simulink model "modulator"  (R2025b)
settings: Solver=ode23tb  StartTime=0.0  StopTime=simlength  FixedStep=tc  MaxStep=tc
undefined symbols (not defined in the file): freq, tc, ts_afe
libraries: SV_pattern_generator_with_global_TRGO x4
settings Model: Creator=dbagn  LastModifiedBy=dbagn
settings SolverCC: NumberNewtonIterations=3.0  ZeroCrossControl=DisableAll  AlgebraicLoopSolver=TrustRegion  SolverResetMethod=Robust
settings DataIOCC: ReturnWorkspaceOutputs=off
settings OptimizationCC: ReuseModelBlockBuffer=off
settings DebuggingCC: UnconnectedInputMsg=warning  UnconnectedOutputMsg=warning  UnconnectedLineMsg=warning
settings ModelReferenceCC: EnableRefExpFcnMdlSchedulingChecks=on
settings SFSimCC: CustomCodeUndefinedFunction=ThrowError
settings SFSimCC: SimCustomHeaderCode=|
  | #include "math_f.h"
  | #include "mavgflt.h"
  | #include "mavgflt_simulink.h"
  | #include "bemf_obsv.h"
  | #include "bemf_obsv_simulink.h"
  | #include "bemf_obsv_load_est.h"
  | #include "bemf_obsv_load_est_simulink.h"
  | #include "dqvector_pi.h"
  | #include "dqvector_pi_simulink.h"
  | #include "sv_pwm_simulink.h"
  | #include "sv_pwm.h"
settings SFSimCC: SimUserSources=|
  | "mavgflt_simulink.c"
  | "mavgflt.c"
  | "bemf_obsv_simulink.c"
  | "bemf_obsv.c"
  | "bemf_obsv_load_est_simulink.c"
  | "bemf_obsv_load_est.c"
  | "dqvector_pi.c"
  | "dqvector_pi_simulink.c"
  | "sv_pwm_simulink.c"
  | "sv_pwm.c"
settings SFSimCC: SimUserIncludeDirs=|
  | include
  | src
settings RTWCC: GPUComputeCapability=3.5  DLArmComputeVersion=19.05

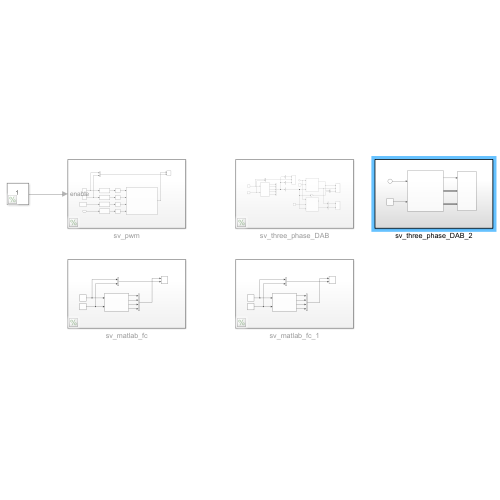
[thumbnail: Simulink's stored preview of the top-level diagram]
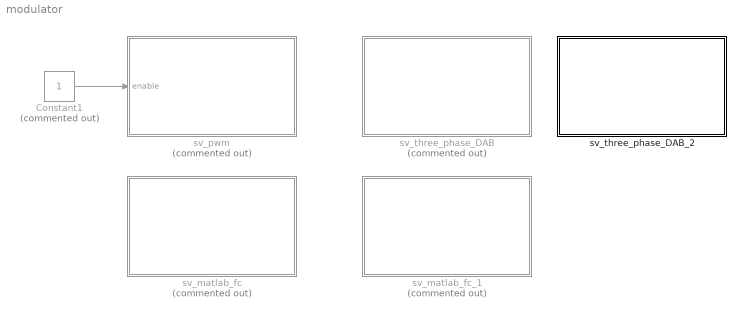
== system modulator ==
  Constant1 : Constant  Commented=on
  sv_matlab_fc : Subsystem  Commented=on
  sv_matlab_fc_1 : Subsystem  Commented=on
  sv_pwm : Subsystem  Commented=on
  sv_three_phase_DAB : Subsystem  Commented=on
  sv_three_phase_DAB_2 : Subsystem
  wires:
  Constant1/1 -> sv_pwm/1(enable)

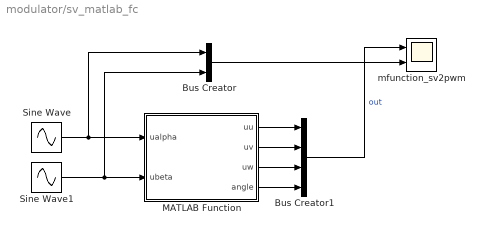
== system modulator/sv_matlab_fc ==
  Bus Creator : BusCreator  Inputs=2
  Bus Creator1 : BusCreator  Inputs=4
  MATLAB Function : MATLAB Function  TreatAsAtomicUnit=on  SystemSampleTime=ts_afe
  Sine Wave : Sin  Amplitude=sqrt(3)/2  Frequency=2*pi*50  SampleTime=0
  Sine Wave1 : Sin  Amplitude=sqrt(3)/2  Frequency=2*pi*50  Phase=-pi/2  SampleTime=0
  mfunction_sv2pwm : Scope  NumInputPorts=2
      settings: ActiveDisplayYMinimum=-3.9269908169872405  ActiveDisplayYMaximum=3.9269908169872392
  wires:
  Bus Creator/1 -> mfunction_sv2pwm/2
  Bus Creator1/1 -> mfunction_sv2pwm/1  "out"
  Sine Wave1/1 -> MATLAB Function/2(ubeta), Bus Creator/2
  Sine Wave/1 -> MATLAB Function/1(ualpha), Bus Creator/1
  MATLAB Function/3(uw) -> Bus Creator1/3
  MATLAB Function/2(uv) -> Bus Creator1/2
  MATLAB Function/1(uu) -> Bus Creator1/1
  MATLAB Function/4(angle) -> Bus Creator1/4

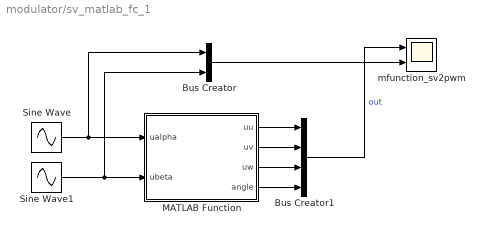
== system modulator/sv_matlab_fc_1 ==
  Bus Creator : BusCreator  Inputs=2
  Bus Creator1 : BusCreator  Inputs=4
  MATLAB Function : MATLAB Function  TreatAsAtomicUnit=on  SystemSampleTime=ts_afe
  Sine Wave : Sin  Amplitude=sqrt(3)/2  Frequency=2*pi*50  SampleTime=0
  Sine Wave1 : Sin  Amplitude=sqrt(3)/2  Frequency=2*pi*50  Phase=-pi/2  SampleTime=0
  mfunction_sv2pwm : Scope  NumInputPorts=2
      settings: ActiveDisplayYMinimum=-0.785398163397448  ActiveDisplayYMaximum=7.0685834705770336
  wires:
  MATLAB Function/4(angle) -> Bus Creator1/4
  MATLAB Function/1(uu) -> Bus Creator1/1
  MATLAB Function/2(uv) -> Bus Creator1/2
  MATLAB Function/3(uw) -> Bus Creator1/3
  Sine Wave/1 -> Bus Creator/1, MATLAB Function/1(ualpha)
  Sine Wave1/1 -> Bus Creator/2, MATLAB Function/2(ubeta)
  Bus Creator1/1 -> mfunction_sv2pwm/1  "out"
  Bus Creator/1 -> mfunction_sv2pwm/2

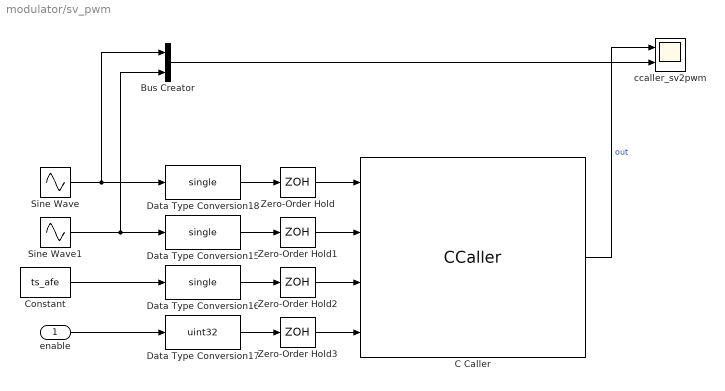
== system modulator/sv_pwm ==
  enable : Inport
  Bus Creator : BusCreator  Inputs=2
  C Caller : CCaller  FunctionName=sv_pwm_process_simulink  PortSpecificationStruct="%)30     .    V @   8    (     @         %    \"     4    !     0         %  0 \"0    $    _    07)G3F%M90  4&]R=$YA;64 4V-O<&4     26YD97@     5'EP90      4VEZ90      27-';&]B86P   X    P    !@    @    $          4    (     0    ,    !         !   P!O=70 #@   #     &    \"     0         !0    @    !     P    $         $  # &]U=  .    .     8    (    !          %    \"     $    &     0         0   ...(+2669 chars)"  SampleTime=ts_afe
  Constant : Constant  Value=ts_afe
  Data Type Conversion15 : DataTypeConversion  OutDataTypeStr=single  SaturateOnIntegerOverflow=off  RndMeth=Floor
  Data Type Conversion16 : DataTypeConversion  OutDataTypeStr=single  SaturateOnIntegerOverflow=off  RndMeth=Floor
  Data Type Conversion17 : DataTypeConversion  OutDataTypeStr=uint32  SaturateOnIntegerOverflow=off  RndMeth=Floor
  Data Type Conversion18 : DataTypeConversion  OutDataTypeStr=single  SaturateOnIntegerOverflow=off  RndMeth=Floor
  Sine Wave : Sin  Amplitude=sqrt(3)/2  Frequency=2*pi*50  SampleTime=0
  Sine Wave1 : Sin  Amplitude=sqrt(3)/2  Frequency=2*pi*50  Phase=pi/2  SampleTime=0
  Zero-Order Hold{,1..3} (4 alike) : ZeroOrderHold  SampleTime=ts_afe
  ccaller_sv2pwm : Scope  NumInputPorts=2
      settings: SampleTime=ts_afe  ActiveDisplayYMinimum=-0.54922  ActiveDisplayYMaximum=1.54922
  wires:
  Zero-Order Hold2/1 -> C Caller/3
  Constant/1 -> Data Type Conversion16/1
  Data Type Conversion18/1 -> Zero-Order Hold/1
  enable/1 -> Data Type Conversion17/1
  Data Type Conversion16/1 -> Zero-Order Hold2/1
  Data Type Conversion17/1 -> Zero-Order Hold3/1
  Zero-Order Hold3/1 -> C Caller/4
  Data Type Conversion15/1 -> Zero-Order Hold1/1
  Zero-Order Hold/1 -> C Caller/1
  Zero-Order Hold1/1 -> C Caller/2
  C Caller/1 -> ccaller_sv2pwm/1  "out"
  Sine Wave/1 -> Bus Creator/1, Data Type Conversion18/1
  Sine Wave1/1 -> Bus Creator/2, Data Type Conversion15/1
  Bus Creator/1 -> ccaller_sv2pwm/2

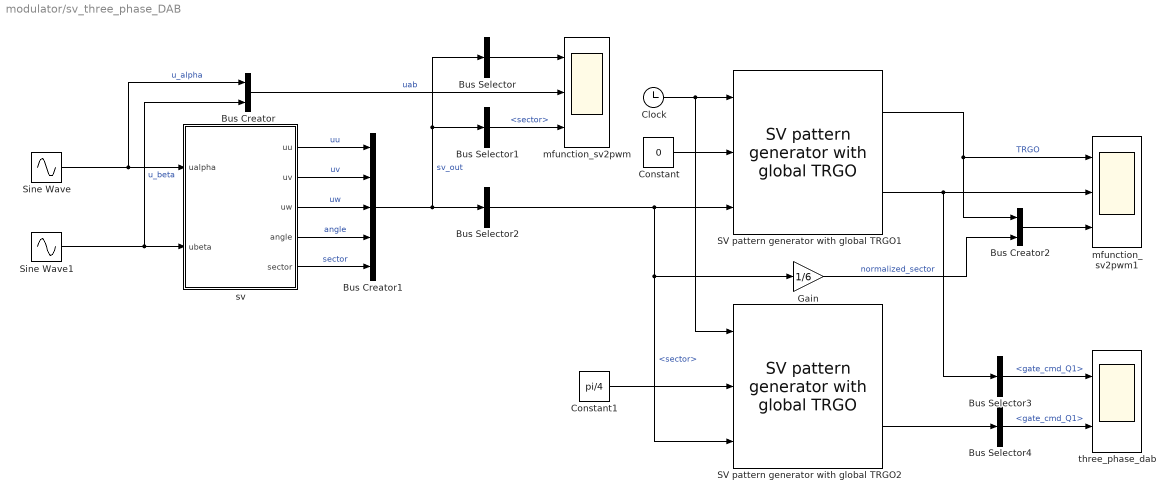
== system modulator/sv_three_phase_DAB ==
  Bus Creator : BusCreator  Inputs=2
  Bus Creator1 : BusCreator  Inputs=5
  Bus Creator2 : BusCreator  Inputs=2
  Bus Selector : BusSelector  OutputSignals=uu,uv,uw,angle  OutputAsBus=on
  Bus Selector1 : BusSelector  OutputSignals=sector
  Bus Selector2 : BusSelector  OutputSignals=sector
  Bus Selector3 : BusSelector  OutputSignals=gate_cmd_Q1
  Bus Selector4 : BusSelector  OutputSignals=gate_cmd_Q1
  Clock : Clock
  Constant : Constant  Value=0
  Constant1 : Constant  Value=pi/4
  Gain : Gain  Gain=1/6
  SV pattern generator with global TRGO1 : SV_pattern_generator_with_global_TRGO/SV pattern generator with global TRGO  f=fPWM_DAB  m_up=0.98  m_low=0.02  dead_time=0  pos_cmd_gate=15  neg_cmd_gate=-10  tc=tc
  SV pattern generator with global TRGO2 : SV_pattern_generator_with_global_TRGO/SV pattern generator with global TRGO  f=fPWM_DAB  m_up=0.98  m_low=0.02  dead_time=0  pos_cmd_gate=15  neg_cmd_gate=-10  tc=tc
  Sine Wave : Sin  Amplitude=sqrt(3)/2  Frequency=2*pi*freq  SampleTime=0
  Sine Wave1 : Sin  Amplitude=sqrt(3)/2  Frequency=2*pi*freq  Phase=-pi/2  SampleTime=0
  mfunction_sv2pwm : Scope  NumInputPorts=3
      settings: ActiveDisplayString=3  ActiveDisplayYMinimum=0.37500000000000022  ActiveDisplayYMaximum=6.625
  mfunction_sv2pwm1 : Scope  NumInputPorts=3
      settings: ActiveDisplayString=3  ActiveDisplayYMinimum=-0.12499999999999997  ActiveDisplayYMaximum=1.125
  sv : MATLAB Function  TreatAsAtomicUnit=on  SystemSampleTime=tc
  three_phase_dab : Scope  NumInputPorts=2
      settings: ActiveDisplayYMinimum=-13.125  ActiveDisplayYMaximum=18.125  DataLoggingVariableName=ScopeData2
  wires:
  Bus Creator/1 -> mfunction_sv2pwm/2  "uab"
  Sine Wave1/1 -> Bus Creator/2, sv/2(ubeta)  "u_beta"
  Sine Wave/1 -> sv/1(ualpha), Bus Creator/1  "u_alpha"
  sv/3(uw) -> Bus Creator1/3  "uw"
  sv/2(uv) -> Bus Creator1/2  "uv"
  sv/1(uu) -> Bus Creator1/1  "uu"
  sv/4(angle) -> Bus Creator1/4  "angle"
  sv/5(sector) -> Bus Creator1/5  "sector"
  Bus Creator1/1 -> Bus Selector2/1, Bus Selector1/1, Bus Selector/1  "sv_out"
  Bus Selector/1 -> mfunction_sv2pwm/1
  Bus Selector1/1 -> mfunction_sv2pwm/3  "<sector>"
  Bus Selector2/1 -> Gain/1, SV pattern generator with global TRGO2/3, SV pattern generator with global TRGO1/3  "<sector>"
  Clock/1 -> SV pattern generator with global TRGO2/1, SV pattern generator with global TRGO1/1
  Constant/1 -> SV pattern generator with global TRGO1/2
  SV pattern generator with global TRGO1/2 -> Bus Selector3/1, mfunction_sv2pwm1/2
  SV pattern generator with global TRGO1/1 -> Bus Creator2/1, mfunction_sv2pwm1/1  "TRGO"
  Bus Creator2/1 -> mfunction_sv2pwm1/3
  Gain/1 -> Bus Creator2/2  "normalized_sector"
  SV pattern generator with global TRGO2/2 -> Bus Selector4/1
  Constant1/1 -> SV pattern generator with global TRGO2/2
  Bus Selector3/1 -> three_phase_dab/1  "<gate_cmd_Q1>"
  Bus Selector4/1 -> three_phase_dab/2  "<gate_cmd_Q1>"

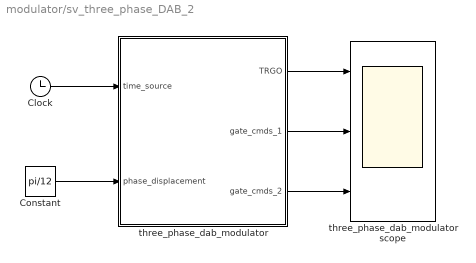
== system modulator/sv_three_phase_DAB_2 ==
  Clock : Clock
  Constant : Constant  Value=pi/12
  three_phase_dab_modulator : Subsystem  mask{fpwm=2400, tc=tc}
      mask prompts: fpwm "fpwm (Hz)"; tc "sampling time (s)"
  three_phase_dab_modulator scope : Scope  NumInputPorts=3
      settings: ActiveDisplayString=3  ActiveDisplayYMinimum=-13.125  ActiveDisplayYMaximum=18.125
  wires:
  Clock/1 -> three_phase_dab_modulator/1(time_source)
  Constant/1 -> three_phase_dab_modulator/2(phase_displacement)
  three_phase_dab_modulator/1(TRGO) -> three_phase_dab_modulator scope/1
  three_phase_dab_modulator/3(gate_cmds_2) -> three_phase_dab_modulator scope/3
  three_phase_dab_modulator/2(gate_cmds_1) -> three_phase_dab_modulator scope/2

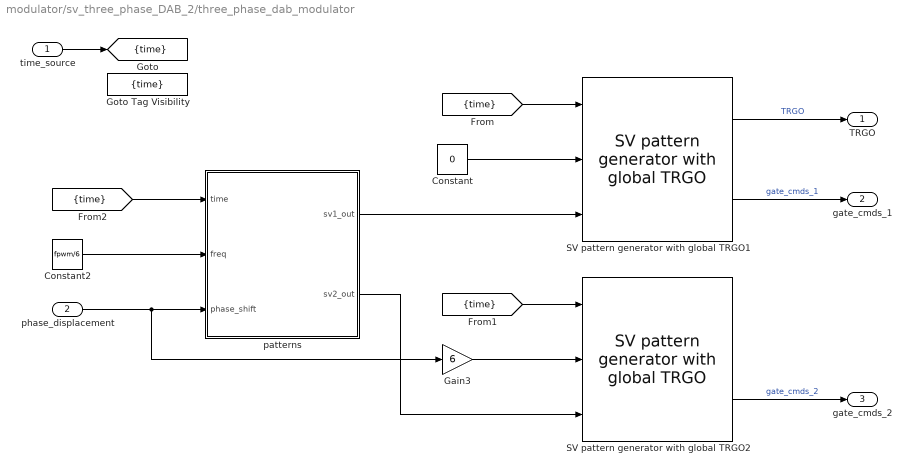
== system modulator/sv_three_phase_DAB_2/three_phase_dab_modulator ==
  time_source : Inport
  phase_displacement : Inport  Port=2
  Constant : Constant  Value=0
  Constant2 : Constant  Value=fpwm/6
  Gain3 : Gain  Gain=6
  Goto Tag Visibility : GotoTagVisibility  GotoTag=time
  SV pattern generator with global TRGO1 : SV_pattern_generator_with_global_TRGO/SV pattern generator with global TRGO  f=fpwm  m_up=0.98  m_low=0.02  dead_time=0  pos_cmd_gate=15  neg_cmd_gate=-10  tc=tc
  SV pattern generator with global TRGO2 : SV_pattern_generator_with_global_TRGO/SV pattern generator with global TRGO  f=fpwm  m_up=0.98  m_low=0.02  dead_time=0  pos_cmd_gate=15  neg_cmd_gate=-10  tc=tc
  patterns : Subsystem
  TRGO : Outport
  gate_cmds_1 : Outport  Port=2
  gate_cmds_2 : Outport  Port=3
  tag scope: time=scoped
  wires:
  SV pattern generator with global TRGO1/2 -> gate_cmds_1/1  "gate_cmds_1"
  Gain3/1 -> SV pattern generator with global TRGO2/2
  Constant/1 -> SV pattern generator with global TRGO1/2
  Constant2/1 -> patterns/2(freq)
  patterns/2(sv2_out) -> SV pattern generator with global TRGO2/3
  patterns/1(sv1_out) -> SV pattern generator with global TRGO1/3
  SV pattern generator with global TRGO1/1 -> TRGO/1  "TRGO"
  phase_displacement/1 -> Gain3/1, patterns/3(phase_shift)
  SV pattern generator with global TRGO2/2 -> gate_cmds_2/1  "gate_cmds_2"
  time_source/1 -> [time]
  [time] -> SV pattern generator with global TRGO1/1
  [time] -> SV pattern generator with global TRGO2/1
  [time] -> patterns/1(time)

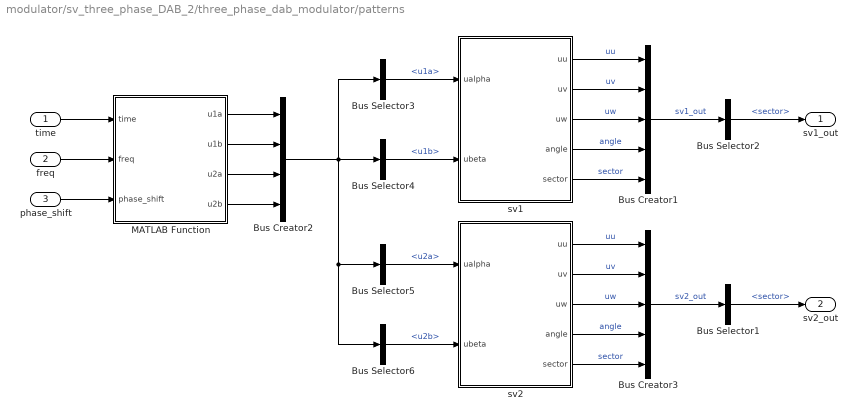
== system modulator/sv_three_phase_DAB_2/three_phase_dab_modulator/patterns ==
  time : Inport
  freq : Inport  Port=2
  phase_shift : Inport  Port=3
  Bus Creator1 : BusCreator  Inputs=5
  Bus Creator2 : BusCreator  Inputs=4
  Bus Creator3 : BusCreator  Inputs=5
  Bus Selector1 : BusSelector  OutputSignals=sector
  Bus Selector2 : BusSelector  OutputSignals=sector
  Bus Selector3 : BusSelector  OutputSignals=u1a
  Bus Selector4 : BusSelector  OutputSignals=u1b
  Bus Selector5 : BusSelector  OutputSignals=u2a
  Bus Selector6 : BusSelector  OutputSignals=u2b
  MATLAB Function : MATLAB Function  TreatAsAtomicUnit=on  SystemSampleTime=tc
  sv1 : MATLAB Function  TreatAsAtomicUnit=on  SystemSampleTime=tc
  sv2 : MATLAB Function  TreatAsAtomicUnit=on  SystemSampleTime=tc
  sv1_out : Outport
  sv2_out : Outport  Port=2
  wires:
  sv2/5(sector) -> Bus Creator3/5  "sector"
  Bus Selector6/1 -> sv2/2(ubeta)  "<u2b>"
  Bus Selector5/1 -> sv2/1(ualpha)  "<u2a>"
  sv2/3(uw) -> Bus Creator3/3  "uw"
  sv1/3(uw) -> Bus Creator1/3  "uw"
  sv2/2(uv) -> Bus Creator3/2  "uv"
  sv2/1(uu) -> Bus Creator3/1  "uu"
  sv2/4(angle) -> Bus Creator3/4  "angle"
  Bus Selector3/1 -> sv1/1(ualpha)  "<u1a>"
  sv1/4(angle) -> Bus Creator1/4  "angle"
  sv1/1(uu) -> Bus Creator1/1  "uu"
  Bus Selector4/1 -> sv1/2(ubeta)  "<u1b>"
  sv1/5(sector) -> Bus Creator1/5  "sector"
  sv1/2(uv) -> Bus Creator1/2  "uv"
  Bus Creator1/1 -> Bus Selector2/1  "sv1_out"
  Bus Selector2/1 -> sv1_out/1  "<sector>"
  Bus Creator3/1 -> Bus Selector1/1  "sv2_out"
  Bus Selector1/1 -> sv2_out/1  "<sector>"
  phase_shift/1 -> MATLAB Function/3(phase_shift)
  time/1 -> MATLAB Function/1(time)
  freq/1 -> MATLAB Function/2(freq)
  MATLAB Function/4(u2b) -> Bus Creator2/4
  MATLAB Function/3(u2a) -> Bus Creator2/3
  MATLAB Function/2(u1b) -> Bus Creator2/2
  MATLAB Function/1(u1a) -> Bus Creator2/1
  Bus Creator2/1 -> Bus Selector3/1, Bus Selector4/1, Bus Selector6/1, Bus Selector5/1

== matlab function modulator/sv_matlab_fc_1/MATLAB Function ==
  data: ualpha input; uu output; ubeta input; uv output; uw output; angle output
function [uu, uv, uw, angle] = sv(ualpha, ubeta)
% SV: Space Vector duty calculation from Clarke (alpha,beta)
% Inputs: ualpha, ubeta  (assumed normalized to reference)
% Outputs: uu,uv,uw (phase duty ratios 0..1), angle (0..2*pi)

% compute angle in [0,2*pi)
angle = mod(atan2(ubeta, ualpha), 2*pi);

% sector 1..6
sector = floor(angle / (pi/3)) + 1;
if sector > 6, sector = 6; end

% compute t1, t2 for each sector (explicitly)
switch sector
    case 1  % 0 .. pi/3
        t1 =  ualpha - ubeta/sqrt(3);    % v1 contribution
        t2 =  2*ubeta/sqrt(3);           % v2 contribution
    case 2  % pi/3 .. 2*pi/3
        t1 = -ualpha + ubeta/sqrt(3);    % v3
        t2 =  ualpha + ubeta/sqrt(3);    % v2
    case 3  % 2*pi/3 .. pi
        t1 =  2*ubeta/sqrt(3);           % v3
        t2 = -ualpha - ubeta/sqrt(3);    % v4
    case 4  % pi .. 4*pi/3
        t1 = -2*ubeta/sqrt(3);           % v5
        t2 =  ubeta/sqrt(3) - ualpha;    % v4
    case 5  % 4*pi/3 .. 5*pi/3
        t1 = -ualpha - ubeta/sqrt(3);    % v5
        t2 =  ualpha - ubeta/sqrt(3);    % v6
    case 6  % 5*pi/3 .. 2*pi
        t1 =  ualpha + ubeta/sqrt(3);    % v1
        t2 = -2*ubeta/sqrt(3);           % v6
    otherwise
        t1 = 0; t2 = 0;
end

% safety: ensure t1,t2 are non-negative in pathological inputs
% (these expressions can be negative depending on ualpha/ubeta signs;
%  we rely on sector selection to produce correct relative signs, but
%  still protect t0 below)
% compute t0
t0 = 1 - (t1 + t2);

% if t0 is negative, scale t1,t2 so that t0 = 0 (avoid negative dwell)
if t0 < 0
    s = 1 / (t1 + t2);    % scale to make t1+t2 == 1
    t1 = t1 * s;
    t2 = t2 * s;
    t0 = 0;
end

% compute phase duty values according to sector mapping
switch sector
    case 1
        ua = t0/2;
        ub = ua + t1;
        uc = ub + t2;
    case 2
        ub = t0/2;
        ua = ub + t1;
        uc = ua + t2;
    case 3
        ub = t0/2;
        uc = ub + t1;
        ua = uc + t2;
    case 4
        uc = t0/2;
        ub = uc + t1;
        ua = ub + t2;
    case 5
        uc = t0/2;
        ua = uc + t1;
        ub = ua + t2;
    case 6
        ua = t0/2;
        uc = ua + t1;
        ub = uc + t2;
    otherwise
        ua = 0; ub = 0; uc = 0;
end

% output
uu = ua;
uv = ub;
uw = uc;
end

== matlab function modulator/sv_matlab_fc/MATLAB Function ==
  data: ualpha input; uu output; ubeta input; uv output; uw output; angle output
function [uu, uv, uw, angle] = sv(ualpha, ubeta)

persistent ua ub uc t0 t1 t2;
if isempty(ua)
    ua = 0;
    ub = 0;
    uc = 0;
    t0 = 0;
    t1 = 0;
    t2 = 0;
end
    angle = atan2(ubeta,ualpha);
    
    if (angle >= 0 && angle <= pi/3)
        % sector1 (counterclockwise)
        t2 = ubeta*2/sqrt(3); %v2
        t1 = ualpha - ubeta/sqrt(3); %v1
        t0 = 1 - t2 - t1;
        ua = t0/2;
        ub = t1 + ua;
        uc = t2 + ub;
    end
    if (angle >= pi/3 && angle <= 2*pi/3)
        % sector2 (clockwise)
        t1 = -ualpha + ubeta/sqrt(3); %v3
        t2 = ualpha + ubeta/sqrt(3); %v2
        t0 = 1 - t2 - t1;
        ub = t0/2;
        ua = t1 + ub;
        uc = t2 + ua;
    end
    if (angle >= 2*pi/3 && angle <= pi)
        % sector3 (counterclockwise)
        t2 = -ubeta/sqrt(3) - ualpha; %v4
        t1 = ubeta*2/sqrt(3); %v3
        t0 = 1 - t2 - t1;
        ub = t0/2;
        uc = t1 + ub;
        ua = t2 + uc;
    end
    if (angle >= -pi && angle <= -2*pi/3)
        % sector4 (clockwise)
        t1 = -2/sqrt(3)*ubeta; %v5
        t2 = ubeta/sqrt(3) - ualpha; %v4
        t0 = 1 - t2 - t1;
        uc = t0/2;
        ub = t1 + uc;
        ua = t2 + ub;
    end

    if (angle >= -2*pi/3 && angle <= -pi/3)
        % sector5 (counterclockwise)
        t2 = ualpha - 1/sqrt(3)*ubeta; %v6
        t1 = -ualpha - 1/sqrt(3)*ubeta; %v5
        t0 = 1 - t2 - t1;
        uc = t0/2;
        ua = t1 + uc;
        ub = t2 + ua;
    end
    if (angle >= -pi/3 && angle <= 0)
        % sector6 (clockwise)
        t1 = ualpha + ubeta/sqrt(3); %v1
        t2 = -ubeta*2/sqrt(3); %v6
        t0 = 1 - t2 - t1;
        ua = t0/2;
        uc = t1 + ua;
        ub = t2 + uc;
    end

uu = ua;
uv = ub;
uw = uc;

== matlab function modulator/sv_three_phase_DAB/sv ==
  data: ualpha input; uu output; ubeta input; uv output; uw output; angle output; sector output
function [uu, uv, uw, angle, sector] = sv(ualpha, ubeta)
% SV: Space Vector duty calculation from Clarke (alpha,beta)
% Inputs: ualpha, ubeta  (assumed normalized to reference)
% Outputs: uu,uv,uw (phase duty ratios 0..1), angle (0..2*pi)

% compute angle in [0,2*pi)
angle = mod(atan2(ubeta, ualpha), 2*pi);

% sector 1..6
sector = floor(angle / (pi/3)) + 1;
if sector > 6, sector = 6; end

% compute t1, t2 for each sector (explicitly)
switch sector
    case 1  % 0 .. pi/3
        t1 =  ualpha - ubeta/sqrt(3);    % v1 contribution
        t2 =  2*ubeta/sqrt(3);           % v2 contribution
    case 2  % pi/3 .. 2*pi/3
        t1 = -ualpha + ubeta/sqrt(3);    % v3
        t2 =  ualpha + ubeta/sqrt(3);    % v2
    case 3  % 2*pi/3 .. pi
        t1 =  2*ubeta/sqrt(3);           % v3
        t2 = -ualpha - ubeta/sqrt(3);    % v4
    case 4  % pi .. 4*pi/3
        t1 = -2*ubeta/sqrt(3);           % v5
        t2 =  ubeta/sqrt(3) - ualpha;    % v4
    case 5  % 4*pi/3 .. 5*pi/3
        t1 = -ualpha - ubeta/sqrt(3);    % v5
        t2 =  ualpha - ubeta/sqrt(3);    % v6
    case 6  % 5*pi/3 .. 2*pi
        t1 =  ualpha + ubeta/sqrt(3);    % v1
        t2 = -2*ubeta/sqrt(3);           % v6
    otherwise
        t1 = 0; t2 = 0;
end

% safety: ensure t1,t2 are non-negative in pathological inputs
% (these expressions can be negative depending on ualpha/ubeta signs;
%  we rely on sector selection to produce correct relative signs, but
%  still protect t0 below)
% compute t0
t0 = 1 - (t1 + t2);

% if t0 is negative, scale t1,t2 so that t0 = 0 (avoid negative dwell)
if t0 < 0
    s = 1 / (t1 + t2);    % scale to make t1+t2 == 1
    t1 = t1 * s;
    t2 = t2 * s;
    t0 = 0;
end

% compute phase duty values according to sector mapping
switch sector
    case 1
        ua = t0/2;
        ub = ua + t1;
        uc = ub + t2;
    case 2
        ub = t0/2;
        ua = ub + t1;
        uc = ua + t2;
    case 3
        ub = t0/2;
        uc = ub + t1;
        ua = uc + t2;
    case 4
        uc = t0/2;
        ub = uc + t1;
        ua = ub + t2;
    case 5
        uc = t0/2;
        ua = uc + t1;
        ub = ua + t2;
    case 6
        ua = t0/2;
        uc = ua + t1;
        ub = uc + t2;
    otherwise
        ua = 0; ub = 0; uc = 0;
end

% output
uu = ua;
uv = ub;
uw = uc;
end

== matlab function modulator/sv_three_phase_DAB_2/three_phase_dab_modulator/patterns/sv1 ==
  data: ualpha input; uu output; ubeta input; uv output; uw output; angle output; sector output
function [uu, uv, uw, angle, sector] = sv(ualpha, ubeta)
% SV: Space Vector duty calculation from Clarke (alpha,beta)
% Inputs: ualpha, ubeta  (assumed normalized to reference)
% Outputs: uu,uv,uw (phase duty ratios 0..1), angle (0..2*pi)

% compute angle in [0,2*pi)
angle = mod(atan2(ubeta, ualpha), 2*pi);

% sector 1..6
sector = floor(angle / (pi/3)) + 1;
if sector > 6, sector = 6; end

% compute t1, t2 for each sector (explicitly)
switch sector
    case 1  % 0 .. pi/3
        t1 =  ualpha - ubeta/sqrt(3);    % v1 contribution
        t2 =  2*ubeta/sqrt(3);           % v2 contribution
    case 2  % pi/3 .. 2*pi/3
        t1 = -ualpha + ubeta/sqrt(3);    % v3
        t2 =  ualpha + ubeta/sqrt(3);    % v2
    case 3  % 2*pi/3 .. pi
        t1 =  2*ubeta/sqrt(3);           % v3
        t2 = -ualpha - ubeta/sqrt(3);    % v4
    case 4  % pi .. 4*pi/3
        t1 = -2*ubeta/sqrt(3);           % v5
        t2 =  ubeta/sqrt(3) - ualpha;    % v4
    case 5  % 4*pi/3 .. 5*pi/3
        t1 = -ualpha - ubeta/sqrt(3);    % v5
        t2 =  ualpha - ubeta/sqrt(3);    % v6
    case 6  % 5*pi/3 .. 2*pi
        t1 =  ualpha + ubeta/sqrt(3);    % v1
        t2 = -2*ubeta/sqrt(3);           % v6
    otherwise
        t1 = 0; t2 = 0;
end

% safety: ensure t1,t2 are non-negative in pathological inputs
% (these expressions can be negative depending on ualpha/ubeta signs;
%  we rely on sector selection to produce correct relative signs, but
%  still protect t0 below)
% compute t0
t0 = 1 - (t1 + t2);

% if t0 is negative, scale t1,t2 so that t0 = 0 (avoid negative dwell)
if t0 < 0
    s = 1 / (t1 + t2);    % scale to make t1+t2 == 1
    t1 = t1 * s;
    t2 = t2 * s;
    t0 = 0;
end

% compute phase duty values according to sector mapping
switch sector
    case 1
        ua = t0/2;
        ub = ua + t1;
        uc = ub + t2;
    case 2
        ub = t0/2;
        ua = ub + t1;
        uc = ua + t2;
    case 3
        ub = t0/2;
        uc = ub + t1;
        ua = uc + t2;
    case 4
        uc = t0/2;
        ub = uc + t1;
        ua = ub + t2;
    case 5
        uc = t0/2;
        ua = uc + t1;
        ub = ua + t2;
    case 6
        ua = t0/2;
        uc = ua + t1;
        ub = uc + t2;
    otherwise
        ua = 0; ub = 0; uc = 0;
end

% output
uu = ua;
uv = ub;
uw = uc;
end

== matlab function modulator/sv_three_phase_DAB_2/three_phase_dab_modulator/patterns/sv2 ==
  data: ualpha input; uu output; ubeta input; uv output; uw output; angle output; sector output
function [uu, uv, uw, angle, sector] = sv(ualpha, ubeta)
% SV: Space Vector duty calculation from Clarke (alpha,beta)
% Inputs: ualpha, ubeta  (assumed normalized to reference)
% Outputs: uu,uv,uw (phase duty ratios 0..1), angle (0..2*pi)

% compute angle in [0,2*pi)
angle = mod(atan2(ubeta, ualpha), 2*pi);

% sector 1..6
sector = floor(angle / (pi/3)) + 1;
if sector > 6, sector = 6; end

% compute t1, t2 for each sector (explicitly)
switch sector
    case 1  % 0 .. pi/3
        t1 =  ualpha - ubeta/sqrt(3);    % v1 contribution
        t2 =  2*ubeta/sqrt(3);           % v2 contribution
    case 2  % pi/3 .. 2*pi/3
        t1 = -ualpha + ubeta/sqrt(3);    % v3
        t2 =  ualpha + ubeta/sqrt(3);    % v2
    case 3  % 2*pi/3 .. pi
        t1 =  2*ubeta/sqrt(3);           % v3
        t2 = -ualpha - ubeta/sqrt(3);    % v4
    case 4  % pi .. 4*pi/3
        t1 = -2*ubeta/sqrt(3);           % v5
        t2 =  ubeta/sqrt(3) - ualpha;    % v4
    case 5  % 4*pi/3 .. 5*pi/3
        t1 = -ualpha - ubeta/sqrt(3);    % v5
        t2 =  ualpha - ubeta/sqrt(3);    % v6
    case 6  % 5*pi/3 .. 2*pi
        t1 =  ualpha + ubeta/sqrt(3);    % v1
        t2 = -2*ubeta/sqrt(3);           % v6
    otherwise
        t1 = 0; t2 = 0;
end

% safety: ensure t1,t2 are non-negative in pathological inputs
% (these expressions can be negative depending on ualpha/ubeta signs;
%  we rely on sector selection to produce correct relative signs, but
%  still protect t0 below)
% compute t0
t0 = 1 - (t1 + t2);

% if t0 is negative, scale t1,t2 so that t0 = 0 (avoid negative dwell)
if t0 < 0
    s = 1 / (t1 + t2);    % scale to make t1+t2 == 1
    t1 = t1 * s;
    t2 = t2 * s;
    t0 = 0;
end

% compute phase duty values according to sector mapping
switch sector
    case 1
        ua = t0/2;
        ub = ua + t1;
        uc = ub + t2;
    case 2
        ub = t0/2;
        ua = ub + t1;
        uc = ua + t2;
    case 3
        ub = t0/2;
        uc = ub + t1;
        ua = uc + t2;
    case 4
        uc = t0/2;
        ub = uc + t1;
        ua = ub + t2;
    case 5
        uc = t0/2;
        ua = uc + t1;
        ub = ua + t2;
    case 6
        ua = t0/2;
        uc = ua + t1;
        ub = uc + t2;
    otherwise
        ua = 0; ub = 0; uc = 0;
end

% output
uu = ua;
uv = ub;
uw = uc;
end

== matlab function modulator/sv_three_phase_DAB_2/three_phase_dab_modulator/patterns/MATLAB Function ==
  data: time input; u1a output; freq input; phase_shift input; u1b output; u2a output; u2b output
function [u1a,u1b,u2a,u2b] = fcn(time, freq, phase_shift)

u1a = cos(2*pi*freq*time -pi/2);
u1b = sin(2*pi*freq*time -pi/2);
u2a = cos(2*pi*freq*time -pi/2 - phase_shift);
u2b = sin(2*pi*freq*time -pi/2 - phase_shift);
